simulink model "SHRKIM002_Dubins"  (R2026a)
settings: Solver=VariableStepAuto  StopTime=inf  MaxStep=0.04
InitFcn:
  | % Robot params
  | r_w = (67.60 / 2) / 1000; % wheel radius in m
  | d = (83 + 12.5 + 12.5) / 1000; % wheel centre-centre distance (width)
  | a = 33.275 / 1000; % IMU to wheel axle distance
  | 
  | % Motor params
  | k = 0.0192;
  | tau = 0.1718;
  | k_bodge = 3;
  | tau_bodge = 0.4;
  | 
  | noiseScalar = 1;
  | 
  | %control loop update rate
  | dt_loop = 0.02;
  | dt_sim = 0.005;
  | dt_plot = 0.1;
  | 
  | waypoint_matrix = centerlineTrack('SaoPaulo.csv');
model workspace (MAT data in the model file):
  d : Simulink.Parameter (value not decoded)
  dphi_limit : Simulink.Parameter (value not decoded)
  dt_sim : Simulink.Parameter (value not decoded)
  l_robot : Simulink.Parameter (value not decoded)
  m_robot : Simulink.Parameter (value not decoded)
  mpc_comp : object (value not decoded)
  nlobj : nlmpc (value not decoded)
  no_points : Simulink.Parameter (value not decoded)
  r_w : Simulink.Parameter (value not decoded)
  rho_min : Simulink.Parameter (value not decoded)
  robot_half_w : Simulink.Parameter (value not decoded)
  sample_f : Simulink.Parameter (value not decoded)
  track_width : Simulink.Parameter (value not decoded)
  waypoint_gain : Simulink.Parameter (value not decoded)
values from neighbouring files (symbols this model uses):
  dphi_limit = 9.72    [controlNMPC.m]
symbols that are objects in the model workspace (value not decoded): l_robot, m_robot, no_points, rho_min, sample_f, waypoint_gain
undefined symbols (not defined in the file or in its folder): DiscIntNeverNeededParam
libraries: simulink x12, dspstat3 x6, slpidlib x2, mpclib x2, robotalgslib x1
(part 2 of 2)

== matlab function SHRKIM002_Dubins/Robot Navigation & Control/Trajectory Generator/Dubins Trajectory Function ==
  data: Waypoints input; no_points parameter; p_des_array output; pose_est_xy input size=[2 1]; p_des output size=[2 1]; psi_des output size=1; kappa_des output size=1; index output; kappa_max output; dk_max output; n_jumps output; s_des output; v_lim_des output; dphi_limit parameter; sample_f parameter; r_w parameter; d parameter; rho_min parameter; L_actual output; T_pure_cent output; K_tot output
function [p_des_array, p_des, psi_des, kappa_des, index, kappa_max, dk_max, n_jumps, s_des, v_lim_des, L_actual, T_pure_cent, K_tot] = dubins(Waypoints, no_points, pose_est_xy, dphi_limit, sample_f, r_w, d, rho_min)
% Cubic Spline with arc length parameterisation

persistent p_array psi_array kappa_array kmax dkmax nj s_array vlim_array index_prev n_window T_pc Ktot
if isempty(p_array)
    [p_array, psi_array, kappa_array, s_array] = buildtrack(Waypoints, no_points, rho_min);
    % find maximum curvature
    kmax = max(abs(kappa_array));
    dk = abs(diff(kappa_array)); 
    % find biggest jump between neighbouring samples
    dkmax = max(dk);
    nj = sum(dk > 0.5); % jumps larger than 0.5

    ds_seg = diff(s_array);

    % total amount the robot turns over one lap
    Ktot = sum(abs(kappa_array(1:end-1)) .* ds_seg);
    % fastest lap if robot exactly on centerline
    T_pc = (s_array(end) + (d/2)*Ktot)/(r_w*dphi_limit);

    % wheel-sat lim top speed on straight
    v_max_f = r_w*dphi_limit;
    % top speed at each point that keeps outer turning wheel in sat lim 
    v_max_out= v_max_f ./(1 + abs(kappa_array)*d/2);

    Ts = 1/sample_f;
    ds= s_array(end)/(no_points-1);
    % no. of path samples robot can do in one control step at top speed +1
    n_ticks = ceil(v_max_f*Ts/ds) + 1;
    vlim_array = v_max_out;
    for j = 1:no_points
        % last point within reach during step
        j_last = min(j+n_ticks, no_points);
        vmin = v_max_out(j);
        for k = j+1:j_last
            vmin = min(vmin, v_max_out(k));
        end
        % lowest final speed limit before controller updates (so robot slows
        % before taking a corner instead of slows inside the corner)
        vlim_array(j) = vmin;
    end

    index_prev = 1;
    % how many ticks robot should look on either side of point (plus safety margin) 
    n_window    = 5*n_ticks + 10;
end

% upper and lower window so it stays in array
window_lower = max(1, index_prev - n_window);
window_upper = min(no_points, index_prev + n_window);

dmin = inf; 
index = index_prev;
% center of window on last ctrl step's point
% check in window and find closest point's index
for j = window_lower:window_upper
    squ_dist_j = (p_array(1,j)-pose_est_xy(1))^2 + (p_array(2,j)-pose_est_xy(2))^2;
    if squ_dist_j < dmin 
        dmin = squ_dist_j; 
        index = j; 
    end
end

index_prev = index;

p_des = p_array(:, index);
p_des_array = p_array;
psi_des = psi_array(index);
kappa_des = kappa_array(index);
s_des = s_array(index);
v_lim_des = vlim_array(index);
kappa_max = kmax;
dk_max  = dkmax;
n_jumps = nj;
L_actual = s_array(end);
T_pure_cent = T_pc;
K_tot  = Ktot;
end



% build track ahead of time to stop it from constantly rebuilding


function [p, psi, kappa, s_steps] = buildtrack(Waypoints, no_points, rho)

% change step to skip waypoints
wp_step = 1;
Nw = size(Waypoints, 2);
W = Waypoints(:, [1:wp_step:Nw-1, Nw]);
% New number of points to travel through
N = size(W,2);

% heading (psi) at waypoints
h_psi = zeros(1, N);
for i = 1:N
    if i == 1
        t = W(:,2) - W(:,1);
    elseif i == N
        t = W(:,N) - W(:,N-1);
    else
        t = W(:,i+1) - W(:,i-1);
    end
    h_psi(i) = atan2(t(2), t(1));
end

% Shortest Dubin per 3 primitives

K = 3*(N-1);
% signs for directions: L= +1, R = -1, S =0
sgn_K = zeros(1, K);
% primitive length
L_K   = zeros(1, K); 
% primitive start pose
p0_K  = zeros(3, K); 
for i = 1:N-1
    [sg, len] = dubinsLeg(W(:,i), h_psi(i), W(:,i+1), h_psi(i+1), rho);
    % leg starts on its waypoint
    q = [W(:,i); h_psi(i)];  
    for j = 1:3
        k = 3*(i-1) + j; 
        L_K(k)    = len(j);
        % zero length arc, treat as S
        sgn_K(k)  = sg(j)*(len(j) > 1e-12);  
        p0_K(:,k) = q;
        [q, ~] = evalPrim(q, sg(j), len(j), rho);
    end
end
 
% sample whole path at equal arc length steps
s_cum = [0, cumsum(L_K)];
s_steps = linspace(0, s_cum(end), no_points);
 
p = zeros(2, no_points);
psi = zeros(1, no_points);
kappa = zeros(1, no_points);
 
k = 1;
for n = 1:no_points
    while (k < K) && (s_steps(n) > s_cum(k+1))
        k = k + 1;
    end
    s_l = s_steps(n) - s_cum(k);
    [q, kap] = evalPrim(p0_K(:,k), sgn_K(k), s_l, rho);
    p(:,n) = q(1:2);
    % wrap to +/- 180
    psi(n) = atan2(sin(q(3)), cos(q(3)));
    kappa(n) = kap;
end
end
 
 
function [sg_best, le_best] = dubinsLeg(P_s, th_s, P_g, th_g, rho)
 
% goal pose wrt to the start pose
dX  = P_g - P_s;
dx  =  cos(th_s)*dX(1) + sin(th_s)*dX(2);
dy  = -sin(th_s)*dX(1) + cos(th_s)*dX(2);
dth = th_g - th_s;
 
% Turn directions sgn(phi_i) for LSL RSR LSR RSL LRL RLR
S = [ 1  0  1;
     -1  0 -1;
      1  0 -1;
     -1  0  1;
      1 -1  1;
     -1  1 -1];
 
L_best   = inf;
sg_best  = [0 0 0];
le_best = [hypot(dx, dy) 0 0];
 
for w = 1:6
    s1 = S(w,1); 
    s2 = S(w,2); 
    s3 = S(w,3);
    % signed radii
    r1 = s1*rho;  
    r3 = s3*rho; 
 
    % CSC
    % writing excerpt equation numbers included so easier to follow
    if s2 == 0                               
        a  = dx - r3*sin(dth); % (1.7)
        b  = dy - (r1 - r3*cos(dth));
        q2 = a^2 + b^2 - (r3 - r1)^2;
        if q2 < 0 
            continue; 
        end
        dx2 = sqrt(q2); % (1.9)
        theta_d_1  = 2*atan2(dx2 - a, b+r3 - r1); % (1.11)
        theta_d_1  = s1*wrap2pi(s1*theta_d_1); % (1.15)
        theta_d_3  = s3*wrap2pi(s3*(dth - theta_d_1)); % (1.13) and (1.15)
        len = [abs(theta_d_1)*rho, dx2, abs(theta_d_3)*rho];
    
    % CCC
    else
        a  = 0.5*(sin(dth) - dx/r1); % (1.6)
        b  = 0.5*(1 - cos(dth) - dy/r1);
        q2 = a^2 + b^2;
        if q2 > 4 
            continue; 
        end
        theta_d_2 = s1*acos(1 - q2/2); % (1.8)
        theta_d_1 = 2*atan2(s1*sqrt(q2) - a, b) - theta_d_2/2; % (1.10)
        theta_d_1 = s1*wrap2pi(s1*theta_d_1); % (1.14)
        theta_d_2 = s2*wrap2pi(s2*theta_d_2);
        theta_d_3 = s3*wrap2pi(s3*(dth - theta_d_1 - theta_d_2)); % (1.12) and (1.14)
        len = [abs(theta_d_1)*rho, abs(theta_d_2)*rho, abs(theta_d_3)*rho];
    end
 
    if sum(len) < L_best
        L_best   = sum(len);
        sg_best  = [s1 s2 s3];
        le_best = len;
    end
end
end
 
 
function [q, kap] = evalPrim(q_0, sg, s, rho)
% pose after traveling s along one primitive from pose q0
% straight
if sg == 0 
    q = [q_0(1) + s*cos(q_0(3)); q_0(2) + s*sin(q_0(3)); q_0(3)];
    kap = 0;
% arc of signed radius r
else 
    r= sg*rho;
    th= q_0(3) + s/r;
    q = [q_0(1) + r*(sin(th) - sin(q_0(3))); q_0(2) - r*(cos(th)-cos(q_0(3))); th];
    kap = 1/r;
end
end
 
 
function a = wrap2pi(a)
% wrap angle so that when it gets very close to 2pi it wraps around to 0
a = mod(a, 2*pi);
if a > 2*pi - 1e-9
    a = 0;
end
end
